simulink model "mit_simscape_model"  (R2026b)
settings: Solver=FixedStepDiscrete  StopTime=t_stop  FixedStep=T_sample
undefined symbols (not defined in the file or in its folder): B, J, omega_s, P_nom_W, t_step_load
libraries: ee_lib x2, elec_conv_AsynchronousMachineSIUni x1, fl_lib x1, nesl_utility x1
settings Model: Creator=luis  LastModifiedBy=luis
settings SimscapeCC: SimscapeLogType=all  SimscapeNominalValues="[{\"value\":\"1\",\"unit\":\"A\"},{\"value\":\"1\",\"unit\":\"bar\"},{\"value\":\"1\",\"unit\":\"cm^2\"},{\"value\":\"1\",\"unit\":\"cm^3/s\"},{\"value\":\"1\",\"unit\":\"kJ/kg\"},{\"value\":\"1\",\"unit\":\"kW\"},{\"value\":\"1\",\"unit\":\"l\"},{\"value\":\"1\",\"unit\":\"N\"},{\"value\":\"1\",\"unit\":\"N*m\"},{\"value\":\"1\",\"unit\":\"V\"},{\"value\":\"0.001\",\"unit\":\"Wb\"}]"  SimscapeUseEnergyAccounting=off

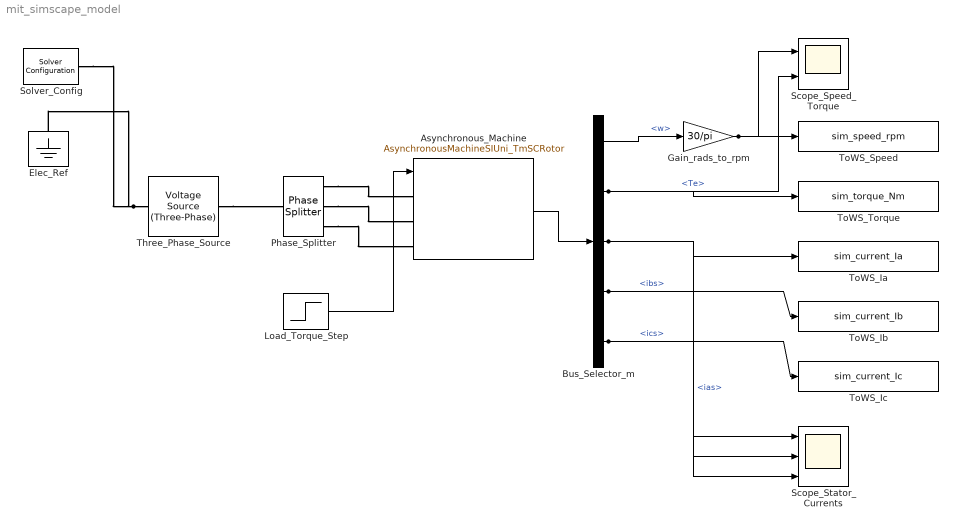
== system mit_simscape_model ==
  Asynchronous_Machine : elec_conv_AsynchronousMachineSIUni/AsynchronousMachineSIUni_TmSCRotor  SRated=P_nom_W  VRated=V_LL_nom  FRated=f_nom  nPolePairs=p_pairs  Rs=R1_Y  Xls=X1_Y  X0=0.9  Rrd=R2_Y  Xlrd=X2_Y  Xm=Xm_Y  Rrd1=0  Xlrd1=0  Rrd2=0  Xlrd2=0  J=J  D=B  saturation_option=ee.enum.saturation.exclude  saturation_i=[0, 4, 9, 18, 25, 34, 50, 68, 95, 120]  saturation_v=[0, 88, 154, 198, 220, 242, 264, 286, 308, 330]  fElectrical0=0  wrm0=0  thm0=0  psids0=0  psiqs0=0  psidr0=0  psiqr0=0  psidr10=0  psiqr10=0  psidr20=0  psiqr20=0  pu2si_i=1  pu2si_v=1  pu2si_wm=omega_s  pu2si_Te=P_nom_W / omega_s  RotorSide_i=0  RotorSide_v=0
  Bus_Selector_m : BusSelector  OutputSignals=w,Te,ias,ibs,ics
  Elec_Ref : fl_lib/Electrical/Electrical Elements/Electrical Reference
  Gain_rads_to_rpm : Gain  Gain=30/pi
  Load_Torque_Step : Step  Time=t_step_load  FinalValue=T_load_step  SampleTime=0
  Phase_Splitter : ee_lib/Connectors & References/Phase Splitter
  Scope_Speed_Torque : Scope  NumInputPorts=2
  Scope_Stator_Currents : Scope  NumInputPorts=3
  Solver_Config : nesl_utility/Solver Configuration  PhysicalDomain=network_engine_domain  SubClassName=solver  LeftPortType=input  RightPortType=generic  Tones=[]  Harmonics=[]  SimulateNoise=off  Profile=off  UseLocalSampling=off  EnableSwitchedLinearOptims=on  FrequencyDomain=off  UseCCode=off  RelTol=0.001  AbsTol=0.001  MinStep=1e-09  ToWorkspace=off  RevertToSquareIcSolve=off  NumHomotopyIterations=100  PhasorMode=off  PhasorModeNumHarmonics=1  ConsistencySolver=NEWTON_XTOL_AFTER_FTOL  CanonicalOrdering=CANONICAL  OptimizeIntermediates=OPTIMIZED  MulticoreSolverChoice=BACKWARD_EULER  IndexReductionMethod=DerivativeReplacement  DoDC=off  ResidualTolerance=1e-09  ConsistencyTolSource=GLOBAL  ConsistencyAbsTol=0.001  ConsistencyRelTol=0.001  ConsistencyTolFactor=0.001  UseLocalSolver=on  LocalSolverChoice=NE_BACKWARD_EULER_ADVANCER  ResolveIndetEquations=on  FunctionEvalNumThread=1  LocalSolverSampleTime=T_sample  DoFixedCost=off  MaxNonlinIter=3  MaxModeIter=2  ComputeImpulses=off  ImpulseIterations=2  LinearAlgebra=auto  LinearAlgebraNumThread=0  EquationFormulation=NE_TIME_EF  DelaysMemoryBudget=1024  AutomaticFiltering=on  FilteringTimeConstant=0.001  PartitionStorageMethod=AS_NEEDED  PartitionMemoryBudget=1024  PartitionMethod=BALANCED  MultibodyUseLocalSolver=off  MultibodyLocalSolverChoice=ODE1  MultibodyLocalSolverSampleTime=0.001
  Three_Phase_Source : ee_lib/Sources/Voltage Source (Three-Phase)  vline_rms=V_LL_nom V  shift=0 deg  freq=f_nom Hz  impedance_option=1  SShortCircuit=1e6 A*V  XR=15  R=0.01 Ohm  L=3.97e-4 H  harmonic_option=0  harmonic_orders=[5, 7, 11, 13]  harmonic_ratios=[.1, .1, .1, .1]  G_parasitic=0 1/Ohm  I_specify=off  I_priority=None  I=[0, 0, 0] A  I_nominal_specify=off  I_nominal_value=1  I_nominal_unit=A
  ToWS_Ia : ToWorkspace  VariableName=sim_current_Ia  SaveFormat=Timeseries  SampleTime=-1
  ToWS_Ib : ToWorkspace  VariableName=sim_current_Ib  SaveFormat=Timeseries  SampleTime=-1
  ToWS_Ic : ToWorkspace  VariableName=sim_current_Ic  SaveFormat=Timeseries  SampleTime=-1
  ToWS_Speed : ToWorkspace  VariableName=sim_speed_rpm  SaveFormat=Timeseries  SampleTime=-1
  ToWS_Torque : ToWorkspace  VariableName=sim_torque_Nm  SaveFormat=Timeseries  SampleTime=-1
  wires:
  Load_Torque_Step/1 -> Asynchronous_Machine/1
  Asynchronous_Machine/1 -> Bus_Selector_m/1
  Bus_Selector_m/1 -> Gain_rads_to_rpm/1  "<w>"
  Gain_rads_to_rpm/1 -> ToWS_Speed/1, Scope_Speed_Torque/1
  Bus_Selector_m/2 -> ToWS_Torque/1, Scope_Speed_Torque/2  "<Te>"
  Bus_Selector_m/3 -> ToWS_Ia/1, Scope_Stator_Currents/1  "<ias>"
  Bus_Selector_m/4 -> ToWS_Ib/1, Scope_Stator_Currents/2  "<ibs>"
  Bus_Selector_m/5 -> ToWS_Ic/1, Scope_Stator_Currents/3  "<ics>"
  connections:
  Three_Phase_Source/LConn1 -- Solver_Config/RConn1 -- Elec_Ref/LConn1
  Three_Phase_Source/RConn1 -- Phase_Splitter/LConn1
  Phase_Splitter/RConn1 -- Asynchronous_Machine/LConn1
  Phase_Splitter/RConn2 -- Asynchronous_Machine/LConn2
  Phase_Splitter/RConn3 -- Asynchronous_Machine/LConn3
